simulink model "tsc_lazo_cerrado"  (R2024a)
settings: Solver=ode15s  StartTime=0.0  StopTime=tm_final  MaxStep=tm_h  RelTol=1e-9  AbsTol=1e-11
model workspace (MAT data in the model file):
  tm_C1 = 1.87501784269e-05
  tm_C2 = 3.75003568539e-05
  tm_Cp = 2.89288467158e-06
  tm_L1 = 0.26018031666
  tm_L2 = 0.13009015833
  tm_R1 = 1.15690788571
  tm_R2 = 0.578453942857
  tm_Rb1 = 84640
  tm_Rb2 = 42320
  tm_Rp = 2.20064
  tm_a1 = 1
  tm_a2 = 0.03
  tm_a3 = 0.03
  tm_carga = [0 1e-05 2e-05 3e-05 4e-05 5e-05 6e-05 7e-05 8e-05 9e-05 0.0001 0.00011 ... (160002 elements, 80001x2)]
  tm_final = 0.8
  tm_h = 2.5e-05
  tm_lambda = 229.793279031
  tm_omega = 314.159265359
  tm_vC10 = 0
  tm_vC20 = 0
  tm_vCp0 = 344.473571203
  tsc_cfg : object (value not decoded)
symbols that are objects in the model workspace (value not decoded): tsc_cfg
(part 2 of 2)

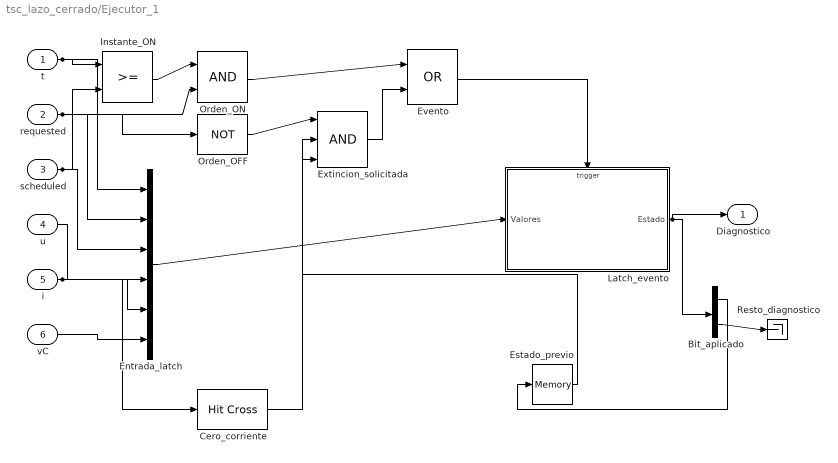
== system tsc_lazo_cerrado/Ejecutor_1 ==
  t : Inport
  requested : Inport  Port=2
  scheduled : Inport  Port=3
  u : Inport  Port=4
  i : Inport  Port=5
  vC : Inport  Port=6
  Bit_aplicado : Demux  Outputs=[1 9]
  Cero_corriente : HitCross
  Entrada_latch : Mux  Inputs=6
  Estado_previo : Memory
  Evento : Logic  Operator=OR  AllPortsSameDT=off  OutDataTypeStr=boolean
  Extincion_solicitada : Logic  Inputs=3  AllPortsSameDT=off  OutDataTypeStr=boolean
  Instante_ON : RelationalOperator  OutDataTypeStr=boolean  RndMeth=Simplest  InputSameDT=off
  Latch_evento : Subsystem
  Orden_OFF : Logic  Operator=NOT  Inputs=1  AllPortsSameDT=off  OutDataTypeStr=boolean
  Orden_ON : Logic  AllPortsSameDT=off  OutDataTypeStr=boolean
  Resto_diagnostico : Terminator
  Diagnostico : Outport
  wires:
  t/1 -> Entrada_latch/1, Instante_ON/1
  requested/1 -> Entrada_latch/2, Orden_ON/2, Orden_OFF/1
  scheduled/1 -> Entrada_latch/3, Instante_ON/2
  u/1 -> Entrada_latch/4
  i/1 -> Entrada_latch/5, Cero_corriente/1
  vC/1 -> Entrada_latch/6
  Instante_ON/1 -> Orden_ON/1
  Orden_OFF/1 -> Extincion_solicitada/1
  Cero_corriente/1 -> Extincion_solicitada/2
  Estado_previo/1 -> Extincion_solicitada/3
  Orden_ON/1 -> Evento/1
  Extincion_solicitada/1 -> Evento/2
  Evento/1 -> Latch_evento/Trigger
  Entrada_latch/1 -> Latch_evento/1(Valores)
  Latch_evento/1(Estado) -> Diagnostico/1, Bit_aplicado/1
  Bit_aplicado/1 -> Estado_previo/1
  Bit_aplicado/2 -> Resto_diagnostico/1

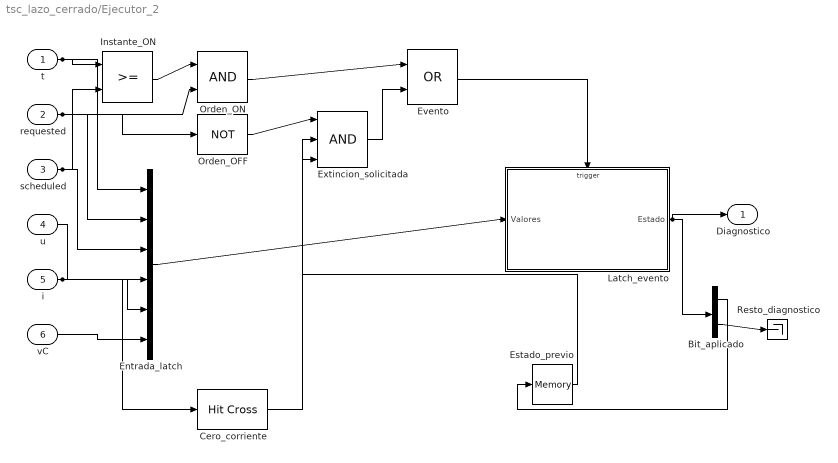
== system tsc_lazo_cerrado/Ejecutor_2 ==
  t : Inport
  requested : Inport  Port=2
  scheduled : Inport  Port=3
  u : Inport  Port=4
  i : Inport  Port=5
  vC : Inport  Port=6
  Bit_aplicado : Demux  Outputs=[1 9]
  Cero_corriente : HitCross
  Entrada_latch : Mux  Inputs=6
  Estado_previo : Memory
  Evento : Logic  Operator=OR  AllPortsSameDT=off  OutDataTypeStr=boolean
  Extincion_solicitada : Logic  Inputs=3  AllPortsSameDT=off  OutDataTypeStr=boolean
  Instante_ON : RelationalOperator  OutDataTypeStr=boolean  RndMeth=Simplest  InputSameDT=off
  Latch_evento : Subsystem
  Orden_OFF : Logic  Operator=NOT  Inputs=1  AllPortsSameDT=off  OutDataTypeStr=boolean
  Orden_ON : Logic  AllPortsSameDT=off  OutDataTypeStr=boolean
  Resto_diagnostico : Terminator
  Diagnostico : Outport
  wires:
  t/1 -> Entrada_latch/1, Instante_ON/1
  requested/1 -> Entrada_latch/2, Orden_ON/2, Orden_OFF/1
  scheduled/1 -> Entrada_latch/3, Instante_ON/2
  u/1 -> Entrada_latch/4
  i/1 -> Entrada_latch/5, Cero_corriente/1
  vC/1 -> Entrada_latch/6
  Instante_ON/1 -> Orden_ON/1
  Orden_OFF/1 -> Extincion_solicitada/1
  Cero_corriente/1 -> Extincion_solicitada/2
  Estado_previo/1 -> Extincion_solicitada/3
  Orden_ON/1 -> Evento/1
  Extincion_solicitada/1 -> Evento/2
  Evento/1 -> Latch_evento/Trigger
  Entrada_latch/1 -> Latch_evento/1(Valores)
  Latch_evento/1(Estado) -> Diagnostico/1, Bit_aplicado/1
  Bit_aplicado/1 -> Estado_previo/1
  Bit_aplicado/2 -> Resto_diagnostico/1

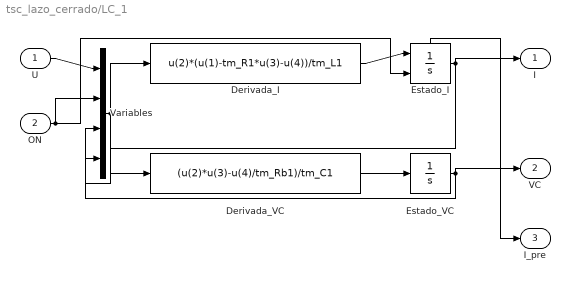
== system tsc_lazo_cerrado/LC_1 ==
  U : Inport
  ON : Inport  Port=2
  Derivada_I : Fcn  Expr=u(2)*(u(1)-tm_R1*u(3)-u(4))/tm_L1
  Derivada_VC : Fcn  Expr=(u(2)*u(3)-u(4)/tm_Rb1)/tm_C1
  Estado_I : Integrator  ExternalReset=falling  ShowStatePort=on
  Estado_VC : Integrator  InitialCondition=tm_vC10
  Variables : Mux
  I : Outport
  VC : Outport  Port=2
  I_pre : Outport  Port=3
  wires:
  U/1 -> Variables/1
  ON/1 -> Variables/2, Estado_I/2
  Estado_I/1 -> Variables/3, I/1
  Estado_VC/1 -> Variables/4, VC/1
  Variables/1 -> Derivada_I/1, Derivada_VC/1
  Derivada_I/1 -> Estado_I/1
  Derivada_VC/1 -> Estado_VC/1
  Estado_I/State -> I_pre/1

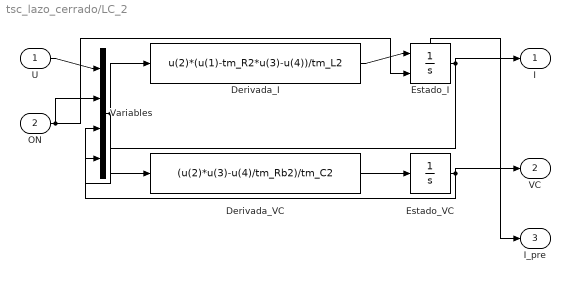
== system tsc_lazo_cerrado/LC_2 ==
  U : Inport
  ON : Inport  Port=2
  Derivada_I : Fcn  Expr=u(2)*(u(1)-tm_R2*u(3)-u(4))/tm_L2
  Derivada_VC : Fcn  Expr=(u(2)*u(3)-u(4)/tm_Rb2)/tm_C2
  Estado_I : Integrator  ExternalReset=falling  ShowStatePort=on
  Estado_VC : Integrator  InitialCondition=tm_vC20
  Variables : Mux
  I : Outport
  VC : Outport  Port=2
  I_pre : Outport  Port=3
  wires:
  U/1 -> Variables/1
  ON/1 -> Variables/2, Estado_I/2
  Estado_I/1 -> Variables/3, I/1
  Estado_VC/1 -> Variables/4, VC/1
  Variables/1 -> Derivada_I/1, Derivada_VC/1
  Derivada_I/1 -> Estado_I/1
  Derivada_VC/1 -> Estado_VC/1
  Estado_I/State -> I_pre/1

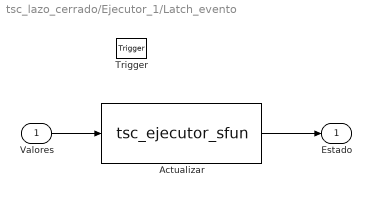
== system tsc_lazo_cerrado/Ejecutor_1/Latch_evento ==
  Valores : Inport
  Trigger : TriggerPort  VariantControl=(inherit)  PortDimensions=1
  Actualizar : M-S-Function  FunctionName=tsc_ejecutor_sfun  Parameters=[tm_L1 tm_R1 tsc_cfg.p.limiteDiDt_A_s tm_vC10]
  Estado : Outport  InitialOutput=[0;-1e6;-1e6;0;0;0;0;0;0;0]
  wires:
  Valores/1 -> Actualizar/1
  Actualizar/1 -> Estado/1

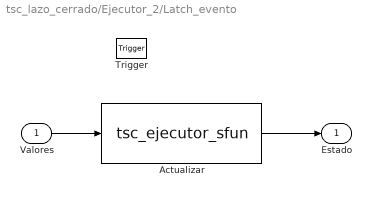
== system tsc_lazo_cerrado/Ejecutor_2/Latch_evento ==
  Valores : Inport
  Trigger : TriggerPort  VariantControl=(inherit)  PortDimensions=1
  Actualizar : M-S-Function  FunctionName=tsc_ejecutor_sfun  Parameters=[tm_L2 tm_R2 tsc_cfg.p.limiteDiDt_A_s tm_vC20]
  Estado : Outport  InitialOutput=[0;-1e6;-1e6;0;0;0;0;0;0;0]
  wires:
  Valores/1 -> Actualizar/1
  Actualizar/1 -> Estado/1
